simulink model "untitled"  (R2025b)
settings: Solver=VariableStepAuto  StartTime=0.0  StopTime=26  RelTol=1e-3
libraries: neural x35
(part 1 of 2)
settings Model: Creator=Jimmy  LastModifiedBy=Pushkaraj
settings DebuggingCC: UnconnectedInputMsg=warning  UnconnectedOutputMsg=warning  UnconnectedLineMsg=warning
settings ModelReferenceCC: EnableRefExpFcnMdlSchedulingChecks=on
settings RTWCC: GPUComputeCapability=3.5  DLArmComputeVersion=19.05

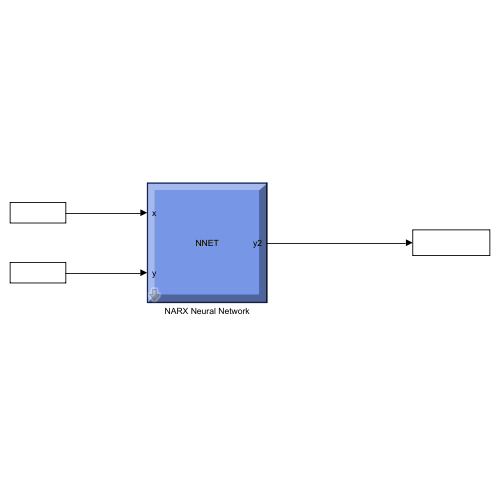
[thumbnail: Simulink's stored preview of the top-level diagram]
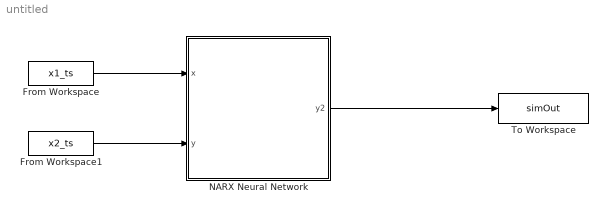
== system untitled ==
  From Workspace : FromWorkspace  VariableName=x1_ts  SampleTime=1  OutputAfterFinalValue=Setting to zero
  From Workspace1 : FromWorkspace  VariableName=x2_ts  SampleTime=1  OutputAfterFinalValue=Setting to zero
  NARX Neural Network : Subsystem  mask{pi_input_1_delayed_1=[0;0;0;0], pi_input_1_delayed_2=[0;0;0;0], pi_input_2_delayed_1=[0;0;0;0;0;0;0;0;0;0], pi_input_2_delayed_2=[0;0;0;0;0;0;0;0;0;0]}
      mask prompts: pi_input_1_delayed_1 "Preprocessed initial input 1 state at timestep 0."; pi_input_1_delayed_2 "Preprocessed initial input 1 state at timestep -1."; pi_input_2_delayed_1 "Preprocessed initial input 2 state at timestep 0."; pi_input_2_delayed_2 "Preprocessed initial input 2 state at timestep -1."
      mask help: NARX Neural Network
      mask Display: e = 0.06;c1 = [120 150 230]/255;c2 = ([120 150 230]+0)/383;c3 = ([120 150 230]+128)/383;patch([0 1 1 0],[0 0 1 1],c1);patch([0 1 1 1-e 1-e 0+e],[0 0 1 1-e 0+e 0+e],c2);patch([0 0 1 1-e 0+e 0+e],[0 1 1 1-e 1-e 0+e],c3);plot([0 1 1 0 0],[0 0 1 1 0]);fprintf('NNET');port_label('input',1,' x');port_label('input',2,' y');port_label('output',1,'y2 ');
  To Workspace : ToWorkspace  VariableName=simOut  SampleTime=-1
  wires:
  From Workspace/1 -> NARX Neural Network/1(x)
  From Workspace1/1 -> NARX Neural Network/2(y)
  NARX Neural Network/1(y2) -> To Workspace/1

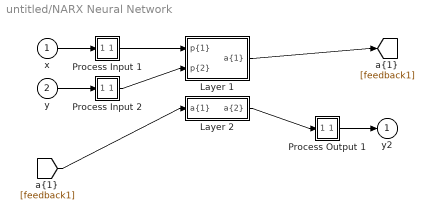
== system untitled/NARX Neural Network ==
  x : Inport  PortDimensions=4  SampleTime=1
      mask Display: e = 0.06;c1 = [120 230 180]/255;c2 = ([120 230 180]+0)/(256+128);c3 = ([120 230 180]+128)/(256+128);patch([0 1 1 0],[0 0 1 1],c1);patch([0 1 1 1-e 1-e 0+e],[0 0 1 1-e 0+e 0+e],c2);patch([0 0 1 1-e 0+e 0+e],[0 1 1 1-e 1-e 0+e],c3);plot([0 1 1 0 0],[0 0 1 1 0]);
  y : Inport  Port=2  PortDimensions=10  SampleTime=1
      mask Display: e = 0.06;c1 = [120 230 180]/255;c2 = ([120 230 180]+0)/(256+128);c3 = ([120 230 180]+128)/(256+128);patch([0 1 1 0],[0 0 1 1],c1);patch([0 1 1 1-e 1-e 0+e],[0 0 1 1-e 0+e 0+e],c2);patch([0 0 1 1-e 0+e 0+e],[0 1 1 1-e 1-e 0+e],c3);plot([0 1 1 0 0],[0 0 1 1 0]);
  Layer 1 : Subsystem
      mask Display: e = 0.06;c1 = [120 150 230]/255;c2 = ([120 150 230]+0)/383;c3 = ([120 150 230]+128)/383;patch([0 1 1 0],[0 0 1 1],c1);patch([0 1 1 1-e 1-e 0+e],[0 0 1 1-e 0+e 0+e],c2);patch([0 0 1 1-e 0+e 0+e],[0 1 1 1-e 1-e 0+e],c3);plot([0 1 1 0 0],[0 0 1 1 0]);
  Layer 2 : Subsystem
      mask Display: e = 0.06;c1 = [120 150 230]/255;c2 = ([120 150 230]+0)/383;c3 = ([120 150 230]+128)/383;patch([0 1 1 0],[0 0 1 1],c1);patch([0 1 1 1-e 1-e 0+e],[0 0 1 1-e 0+e 0+e],c2);patch([0 0 1 1-e 0+e 0+e],[0 1 1 1-e 1-e 0+e],c3);plot([0 1 1 0 0],[0 0 1 1 0]);
  Process Input 1 : Subsystem
      mask Display: e = 0.06;c1 = [120 150 230]/255;c2 = ([120 150 230]+0)/383;c3 = ([120 150 230]+128)/383;patch([0 1 1 0],[0 0 1 1],c1);patch([0 1 1 1-e 1-e 0+e],[0 0 1 1-e 0+e 0+e],c2);patch([0 0 1 1-e 0+e 0+e],[0 1 1 1-e 1-e 0+e],c3);plot([0 1 1 0 0],[0 0 1 1 0]);
  Process Input 2 : Subsystem
      mask Display: e = 0.06;c1 = [120 150 230]/255;c2 = ([120 150 230]+0)/383;c3 = ([120 150 230]+128)/383;patch([0 1 1 0],[0 0 1 1],c1);patch([0 1 1 1-e 1-e 0+e],[0 0 1 1-e 0+e 0+e],c2);patch([0 0 1 1-e 0+e 0+e],[0 1 1 1-e 1-e 0+e],c3);plot([0 1 1 0 0],[0 0 1 1 0]);
  Process Output 1 : Subsystem
      mask Display: e = 0.06;c1 = [120 150 230]/255;c2 = ([120 150 230]+0)/383;c3 = ([120 150 230]+128)/383;patch([0 1 1 0],[0 0 1 1],c1);patch([0 1 1 1-e 1-e 0+e],[0 0 1 1-e 0+e 0+e],c2);patch([0 0 1 1-e 0+e 0+e],[0 1 1 1-e 1-e 0+e],c3);plot([0 1 1 0 0],[0 0 1 1 0]);
  y2 : Outport  InitialOutput=[0;0;0;0;0;0;0;0;0;0]
      mask Display: e = 0.06;c1 = [120 230 180]/255;c2 = ([120 230 180]+0)/(256+128);c3 = ([120 230 180]+128)/(256+128);patch([0 1 1 0],[0 0 1 1],c1);patch([0 1 1 1-e 1-e 0+e],[0 0 1 1-e 0+e 0+e],c2);patch([0 0 1 1-e 0+e 0+e],[0 1 1 1-e 1-e 0+e],c3);plot([0 1 1 0 0],[0 0 1 1 0]);
  wires:
  x/1 -> Process Input 1/1(x)
  y/1 -> Process Input 2/1(x)
  Process Output 1/1(y) -> y2/1
  Process Input 1/1(p) -> Layer 1/1("p{1}")
  Process Input 2/1(p) -> Layer 1/2("p{2}")
  Layer 1/1("a{1}") -> [feedback1]
  [feedback1] -> Layer 2/1("a{1} ")
  Layer 2/1("a{2}") -> Process Output 1/1(a)

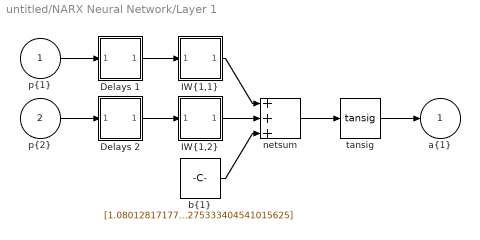
== system untitled/NARX Neural Network/Layer 1 ==
  "p{1}" : Inport  PortDimensions=4  SampleTime=1
      mask Display: e = 0.06;c1 = [120 230 180]/255;c2 = ([120 230 180]+0)/(256+128);c3 = ([120 230 180]+128)/(256+128);patch([0 1 1 0],[0 0 1 1],c1);patch([0 1 1 1-e 1-e 0+e],[0 0 1 1-e 0+e 0+e],c2);patch([0 0 1 1-e 0+e 0+e],[0 1 1 1-e 1-e 0+e],c3);plot([0 1 1 0 0],[0 0 1 1 0]);
  "p{2}" : Inport  Port=2  PortDimensions=10  SampleTime=1
      mask Display: e = 0.06;c1 = [120 230 180]/255;c2 = ([120 230 180]+0)/(256+128);c3 = ([120 230 180]+128)/(256+128);patch([0 1 1 0],[0 0 1 1],c1);patch([0 1 1 1-e 1-e 0+e],[0 0 1 1-e 0+e 0+e],c2);patch([0 0 1 1-e 0+e 0+e],[0 1 1 1-e 1-e 0+e],c3);plot([0 1 1 0 0],[0 0 1 1 0]);
  Delays 1 : Subsystem
      mask Display: e = 0.06;c1 = [120 150 230]/255;c2 = ([120 150 230]+0)/383;c3 = ([120 150 230]+128)/383;patch([0 1 1 0],[0 0 1 1],c1);patch([0 1 1 1-e 1-e 0+e],[0 0 1 1-e 0+e 0+e],c2);patch([0 0 1 1-e 0+e 0+e],[0 1 1 1-e 1-e 0+e],c3);plot([0 1 1 0 0],[0 0 1 1 0]);disp('1-2');
  Delays 2 : Subsystem
      mask Display: e = 0.06;c1 = [120 150 230]/255;c2 = ([120 150 230]+0)/383;c3 = ([120 150 230]+128)/383;patch([0 1 1 0],[0 0 1 1],c1);patch([0 1 1 1-e 1-e 0+e],[0 0 1 1-e 0+e 0+e],c2);patch([0 0 1 1-e 0+e 0+e],[0 1 1 1-e 1-e 0+e],c3);plot([0 1 1 0 0],[0 0 1 1 0]);disp('1-2');
  "IW{1,1}" : Subsystem
      mask Display: e = 0.06;c1 = [120 150 230]/255;c2 = ([120 150 230]+0)/383;c3 = ([120 150 230]+128)/383;patch([0 1 1 0],[0 0 1 1],c1);patch([0 1 1 1-e 1-e 0+e],[0 0 1 1-e 0+e 0+e],c2);patch([0 0 1 1-e 0+e 0+e],[0 1 1 1-e 1-e 0+e],c3);plot([0 1 1 0 0],[0 0 1 1 0]);disp('W');
  "IW{1,2}" : Subsystem
      mask Display: e = 0.06;c1 = [120 150 230]/255;c2 = ([120 150 230]+0)/383;c3 = ([120 150 230]+128)/383;patch([0 1 1 0],[0 0 1 1],c1);patch([0 1 1 1-e 1-e 0+e],[0 0 1 1-e 0+e 0+e],c2);patch([0 0 1 1-e 0+e 0+e],[0 1 1 1-e 1-e 0+e],c3);plot([0 1 1 0 0],[0 0 1 1 0]);disp('W');
  "b{1}" : Constant  Value=[1.0801281717727395648154242735472507774829864501953125;-1.310912600446497489059538565925322473049163818359375;0.9404335907148200224270340186194516718387603759765625;-0.81368279707896140617862101862556301057338714599609375;0.432949116587421134472180028751608915627002716064453125;0.068784327532554534467834628230775706470012664794921875;-0.29264096087120716749296889247489161789417266845703125;0.7805557229172677136119773422251455485820770263671875;-1.12796688888643092951724611339159309864044189453125;1.7338922757099712868011920363642275333404541015625]
      mask Display: e = 0.06;c1 = [120 150 230]/255;c2 = ([120 150 230]+0)/383;c3 = ([120 150 230]+128)/383;patch([0 1 1 0],[0 0 1 1],c1);patch([0 1 1 1-e 1-e 0+e],[0 0 1 1-e 0+e 0+e],c2);patch([0 0 1 1-e 0+e 0+e],[0 1 1 1-e 1-e 0+e],c3);plot([0 1 1 0 0],[0 0 1 1 0]);disp('b');
  netsum : Sum  Inputs=3  InputSameDT=on  SaturateOnIntegerOverflow=on  OutDataTypeStr=Inherit: Same as first input
      mask Display: e = 0.06;c1 = [120 150 230]/255;c2 = ([120 150 230]+0)/383;c3 = ([120 150 230]+128)/383;patch([0 1 1 0],[0 0 1 1],c1);patch([0 1 1 1-e 1-e 0+e],[0 0 1 1-e 0+e 0+e],c2);patch([0 0 1 1-e 0+e 0+e],[0 1 1 1-e 1-e 0+e],c3);plot([0 1 1 0 0],[0 0 1 1 0]);disp('+');
  tansig : neural/Transfer Functions/tansig
  "a{1}" : Outport  InitialOutput=[0;0;0;0;0;0;0;0;0;0]
      mask Display: e = 0.06;c1 = [120 230 180]/255;c2 = ([120 230 180]+0)/(256+128);c3 = ([120 230 180]+128)/(256+128);patch([0 1 1 0],[0 0 1 1],c1);patch([0 1 1 1-e 1-e 0+e],[0 0 1 1-e 0+e 0+e],c2);patch([0 0 1 1-e 0+e 0+e],[0 1 1 1-e 1-e 0+e],c3);plot([0 1 1 0 0],[0 0 1 1 0]);
  wires:
  "p{1}"/1 -> Delays 1/1("p{1}")
  Delays 1/1("pd{1,1}") -> "IW{1,1}"/1("pd{1,1}")
  "IW{1,1}"/1("iz{1,1}") -> netsum/1
  "p{2}"/1 -> Delays 2/1("p{1}")
  Delays 2/1("pd{1,2}") -> "IW{1,2}"/1("pd{1,2}")
  "IW{1,2}"/1("iz{1,2}") -> netsum/2
  "b{1}"/1 -> netsum/3
  netsum/1 -> tansig/1
  tansig/1 -> "a{1}"/1

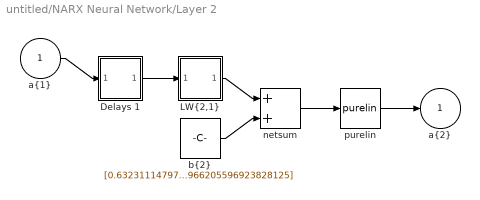
== system untitled/NARX Neural Network/Layer 2 ==
  "a{1} " : Inport  PortDimensions=10  SampleTime=1
      mask Display: e = 0.06;c1 = [120 230 180]/255;c2 = ([120 230 180]+0)/(256+128);c3 = ([120 230 180]+128)/(256+128);patch([0 1 1 0],[0 0 1 1],c1);patch([0 1 1 1-e 1-e 0+e],[0 0 1 1-e 0+e 0+e],c2);patch([0 0 1 1-e 0+e 0+e],[0 1 1 1-e 1-e 0+e],c3);plot([0 1 1 0 0],[0 0 1 1 0]);
  Delays 1 : Subsystem
      mask Display: e = 0.06;c1 = [120 150 230]/255;c2 = ([120 150 230]+0)/383;c3 = ([120 150 230]+128)/383;patch([0 1 1 0],[0 0 1 1],c1);patch([0 1 1 1-e 1-e 0+e],[0 0 1 1-e 0+e 0+e],c2);patch([0 0 1 1-e 0+e 0+e],[0 1 1 1-e 1-e 0+e],c3);plot([0 1 1 0 0],[0 0 1 1 0]);disp('0');
  "LW{2,1}" : Subsystem
      mask Display: e = 0.06;c1 = [120 150 230]/255;c2 = ([120 150 230]+0)/383;c3 = ([120 150 230]+128)/383;patch([0 1 1 0],[0 0 1 1],c1);patch([0 1 1 1-e 1-e 0+e],[0 0 1 1-e 0+e 0+e],c2);patch([0 0 1 1-e 0+e 0+e],[0 1 1 1-e 1-e 0+e],c3);plot([0 1 1 0 0],[0 0 1 1 0]);disp('W');
  "b{2}" : Constant  Value=[0.63231114797012033523770924148266203701496124267578125;0.077425009453641446821592353444430045783519744873046875;0.69336797498678903739488532664836384356021881103515625;0.96191102890088908683452473269426263868808746337890625;-0.01280570802179627383499127546429008361883461475372314453125;0.1820181237505598959014463389394222758710384368896484375;-3.18169363647799041672215025755576789379119873046875;-0.374160373721601657859281431228737346827983856201171875;-0.778234975833982378645714561571367084980010986328125;0.8437778280262862029559300935943610966205596923828125]
      mask Display: e = 0.06;c1 = [120 150 230]/255;c2 = ([120 150 230]+0)/383;c3 = ([120 150 230]+128)/383;patch([0 1 1 0],[0 0 1 1],c1);patch([0 1 1 1-e 1-e 0+e],[0 0 1 1-e 0+e 0+e],c2);patch([0 0 1 1-e 0+e 0+e],[0 1 1 1-e 1-e 0+e],c3);plot([0 1 1 0 0],[0 0 1 1 0]);disp('b');
  netsum : Sum  Inputs=2  InputSameDT=on  SaturateOnIntegerOverflow=on  OutDataTypeStr=Inherit: Same as first input
      mask Display: e = 0.06;c1 = [120 150 230]/255;c2 = ([120 150 230]+0)/383;c3 = ([120 150 230]+128)/383;patch([0 1 1 0],[0 0 1 1],c1);patch([0 1 1 1-e 1-e 0+e],[0 0 1 1-e 0+e 0+e],c2);patch([0 0 1 1-e 0+e 0+e],[0 1 1 1-e 1-e 0+e],c3);plot([0 1 1 0 0],[0 0 1 1 0]);disp('+');
  purelin : neural/Transfer Functions/purelin
  "a{2}" : Outport  InitialOutput=[0;0;0;0;0;0;0;0;0;0]
      mask Display: e = 0.06;c1 = [120 230 180]/255;c2 = ([120 230 180]+0)/(256+128);c3 = ([120 230 180]+128)/(256+128);patch([0 1 1 0],[0 0 1 1],c1);patch([0 1 1 1-e 1-e 0+e],[0 0 1 1-e 0+e 0+e],c2);patch([0 0 1 1-e 0+e 0+e],[0 1 1 1-e 1-e 0+e],c3);plot([0 1 1 0 0],[0 0 1 1 0]);
  wires:
  "a{1} "/1 -> Delays 1/1("p{2}")
  Delays 1/1("pd{2,1}") -> "LW{2,1}"/1("ad{2,1}")
  "LW{2,1}"/1("lz{2,1}") -> netsum/1
  "b{2}"/1 -> netsum/2
  netsum/1 -> purelin/1
  purelin/1 -> "a{2}"/1

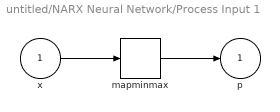
== system untitled/NARX Neural Network/Process Input 1 ==
  x : Inport  PortDimensions=4  SampleTime=1
      mask Display: e = 0.06;c1 = [120 230 180]/255;c2 = ([120 230 180]+0)/(256+128);c3 = ([120 230 180]+128)/(256+128);patch([0 1 1 0],[0 0 1 1],c1);patch([0 1 1 1-e 1-e 0+e],[0 0 1 1-e 0+e 0+e],c2);patch([0 0 1 1-e 0+e 0+e],[0 1 1 1-e 1-e 0+e],c3);plot([0 1 1 0 0],[0 0 1 1 0]);
  mapminmax : neural/Processing Functions/mapminmax  xmin=[0;-4.44000000000000039079850466806;0;0]  xmax=[81;3.33000000000000007105427357601;354;168]  ymin=-1  ymax=1
  p : Outport  PortDimensions=4  SampleTime=1
      mask Display: e = 0.06;c1 = [120 230 180]/255;c2 = ([120 230 180]+0)/(256+128);c3 = ([120 230 180]+128)/(256+128);patch([0 1 1 0],[0 0 1 1],c1);patch([0 1 1 1-e 1-e 0+e],[0 0 1 1-e 0+e 0+e],c2);patch([0 0 1 1-e 0+e 0+e],[0 1 1 1-e 1-e 0+e],c3);plot([0 1 1 0 0],[0 0 1 1 0]);
  wires:
  x/1 -> mapminmax/1
  mapminmax/1 -> p/1

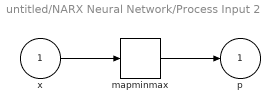
== system untitled/NARX Neural Network/Process Input 2 ==
  x : Inport  PortDimensions=10  SampleTime=1
      mask Display: e = 0.06;c1 = [120 230 180]/255;c2 = ([120 230 180]+0)/(256+128);c3 = ([120 230 180]+128)/(256+128);patch([0 1 1 0],[0 0 1 1],c1);patch([0 1 1 1-e 1-e 0+e],[0 0 1 1-e 0+e 0+e],c2);patch([0 0 1 1-e 0+e 0+e],[0 1 1 1-e 1-e 0+e],c3);plot([0 1 1 0 0],[0 0 1 1 0]);
  mapminmax : neural/Processing Functions/mapminmax  xmin=[0;0;0;0;0;0;0;0;0;0]  xmax=[1;1;1;1;1;1;1;1;1;1]  ymin=-1  ymax=1
  p : Outport  PortDimensions=10  SampleTime=1
      mask Display: e = 0.06;c1 = [120 230 180]/255;c2 = ([120 230 180]+0)/(256+128);c3 = ([120 230 180]+128)/(256+128);patch([0 1 1 0],[0 0 1 1],c1);patch([0 1 1 1-e 1-e 0+e],[0 0 1 1-e 0+e 0+e],c2);patch([0 0 1 1-e 0+e 0+e],[0 1 1 1-e 1-e 0+e],c3);plot([0 1 1 0 0],[0 0 1 1 0]);
  wires:
  x/1 -> mapminmax/1
  mapminmax/1 -> p/1

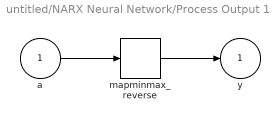
== system untitled/NARX Neural Network/Process Output 1 ==
  a : Inport  PortDimensions=10  SampleTime=1
      mask Display: e = 0.06;c1 = [120 230 180]/255;c2 = ([120 230 180]+0)/(256+128);c3 = ([120 230 180]+128)/(256+128);patch([0 1 1 0],[0 0 1 1],c1);patch([0 1 1 1-e 1-e 0+e],[0 0 1 1-e 0+e 0+e],c2);patch([0 0 1 1-e 0+e 0+e],[0 1 1 1-e 1-e 0+e],c3);plot([0 1 1 0 0],[0 0 1 1 0]);
  mapminmax_reverse : neural/Processing Functions/mapminmax_reverse  xmin=[0;0;0;0;0;0;0;0;0;0]  xmax=[1;1;1;1;1;1;1;1;1;1]  ymin=-1  ymax=1
  y : Outport  PortDimensions=10  SampleTime=1
      mask Display: e = 0.06;c1 = [120 230 180]/255;c2 = ([120 230 180]+0)/(256+128);c3 = ([120 230 180]+128)/(256+128);patch([0 1 1 0],[0 0 1 1],c1);patch([0 1 1 1-e 1-e 0+e],[0 0 1 1-e 0+e 0+e],c2);patch([0 0 1 1-e 0+e 0+e],[0 1 1 1-e 1-e 0+e],c3);plot([0 1 1 0 0],[0 0 1 1 0]);
  wires:
  a/1 -> mapminmax_reverse/1
  mapminmax_reverse/1 -> y/1

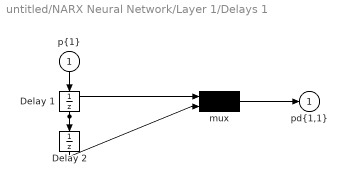
== system untitled/NARX Neural Network/Layer 1/Delays 1 ==
  "p{1}" : Inport  PortDimensions=4  SampleTime=1
      mask Display: e = 0.06;c1 = [120 230 180]/255;c2 = ([120 230 180]+0)/(256+128);c3 = ([120 230 180]+128)/(256+128);patch([0 1 1 0],[0 0 1 1],c1);patch([0 1 1 1-e 1-e 0+e],[0 0 1 1-e 0+e 0+e],c2);patch([0 0 1 1-e 0+e 0+e],[0 1 1 1-e 1-e 0+e],c3);plot([0 1 1 0 0],[0 0 1 1 0]);
  Delay 1 : UnitDelay  InitialCondition=pi_input_1_delayed_1
      mask Display: e = 0.06;c1 = [120 150 230]/255;c2 = ([120 150 230]+0)/383;c3 = ([120 150 230]+128)/383;patch([0 1 1 0],[0 0 1 1],c1);patch([0 1 1 1-e 1-e 0+e],[0 0 1 1-e 0+e 0+e],c2);patch([0 0 1 1-e 0+e 0+e],[0 1 1 1-e 1-e 0+e],c3);plot([0 1 1 0 0],[0 0 1 1 0]);disp('D')
  Delay 2 : UnitDelay  InitialCondition=pi_input_1_delayed_2
      mask Display: e = 0.06;c1 = [120 150 230]/255;c2 = ([120 150 230]+0)/383;c3 = ([120 150 230]+128)/383;patch([0 1 1 0],[0 0 1 1],c1);patch([0 1 1 1-e 1-e 0+e],[0 0 1 1-e 0+e 0+e],c2);patch([0 0 1 1-e 0+e 0+e],[0 1 1 1-e 1-e 0+e],c3);plot([0 1 1 0 0],[0 0 1 1 0]);disp('D')
  mux : Mux  Inputs=2
      mask Display: e = 0.06;c1 = [120 150 230]/255;c2 = ([120 150 230]+0)/383;c3 = ([120 150 230]+128)/383;patch([0 1 1 0],[0 0 1 1],c1);patch([0 1 1 1-e 1-e 0+e],[0 0 1 1-e 0+e 0+e],c2);patch([0 0 1 1-e 0+e 0+e],[0 1 1 1-e 1-e 0+e],c3);plot([0 1 1 0 0],[0 0 1 1 0]);disp('Mux')
  "pd{1,1}" : Outport
      mask Display: e = 0.06;c1 = [120 230 180]/255;c2 = ([120 230 180]+0)/(256+128);c3 = ([120 230 180]+128)/(256+128);patch([0 1 1 0],[0 0 1 1],c1);patch([0 1 1 1-e 1-e 0+e],[0 0 1 1-e 0+e 0+e],c2);patch([0 0 1 1-e 0+e 0+e],[0 1 1 1-e 1-e 0+e],c3);plot([0 1 1 0 0],[0 0 1 1 0]);
  wires:
  "p{1}"/1 -> Delay 1/1
  Delay 1/1 -> Delay 2/1, mux/1
  Delay 2/1 -> mux/2
  mux/1 -> "pd{1,1}"/1

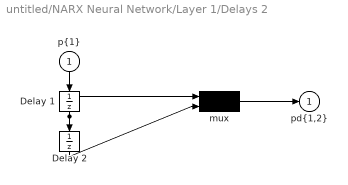
== system untitled/NARX Neural Network/Layer 1/Delays 2 ==
  "p{1}" : Inport  PortDimensions=10  SampleTime=1
      mask Display: e = 0.06;c1 = [120 230 180]/255;c2 = ([120 230 180]+0)/(256+128);c3 = ([120 230 180]+128)/(256+128);patch([0 1 1 0],[0 0 1 1],c1);patch([0 1 1 1-e 1-e 0+e],[0 0 1 1-e 0+e 0+e],c2);patch([0 0 1 1-e 0+e 0+e],[0 1 1 1-e 1-e 0+e],c3);plot([0 1 1 0 0],[0 0 1 1 0]);
  Delay 1 : UnitDelay  InitialCondition=pi_input_2_delayed_1
      mask Display: e = 0.06;c1 = [120 150 230]/255;c2 = ([120 150 230]+0)/383;c3 = ([120 150 230]+128)/383;patch([0 1 1 0],[0 0 1 1],c1);patch([0 1 1 1-e 1-e 0+e],[0 0 1 1-e 0+e 0+e],c2);patch([0 0 1 1-e 0+e 0+e],[0 1 1 1-e 1-e 0+e],c3);plot([0 1 1 0 0],[0 0 1 1 0]);disp('D')
  Delay 2 : UnitDelay  InitialCondition=pi_input_2_delayed_2
      mask Display: e = 0.06;c1 = [120 150 230]/255;c2 = ([120 150 230]+0)/383;c3 = ([120 150 230]+128)/383;patch([0 1 1 0],[0 0 1 1],c1);patch([0 1 1 1-e 1-e 0+e],[0 0 1 1-e 0+e 0+e],c2);patch([0 0 1 1-e 0+e 0+e],[0 1 1 1-e 1-e 0+e],c3);plot([0 1 1 0 0],[0 0 1 1 0]);disp('D')
  mux : Mux  Inputs=2
      mask Display: e = 0.06;c1 = [120 150 230]/255;c2 = ([120 150 230]+0)/383;c3 = ([120 150 230]+128)/383;patch([0 1 1 0],[0 0 1 1],c1);patch([0 1 1 1-e 1-e 0+e],[0 0 1 1-e 0+e 0+e],c2);patch([0 0 1 1-e 0+e 0+e],[0 1 1 1-e 1-e 0+e],c3);plot([0 1 1 0 0],[0 0 1 1 0]);disp('Mux')
  "pd{1,2}" : Outport
      mask Display: e = 0.06;c1 = [120 230 180]/255;c2 = ([120 230 180]+0)/(256+128);c3 = ([120 230 180]+128)/(256+128);patch([0 1 1 0],[0 0 1 1],c1);patch([0 1 1 1-e 1-e 0+e],[0 0 1 1-e 0+e 0+e],c2);patch([0 0 1 1-e 0+e 0+e],[0 1 1 1-e 1-e 0+e],c3);plot([0 1 1 0 0],[0 0 1 1 0]);
  wires:
  "p{1}"/1 -> Delay 1/1
  Delay 1/1 -> Delay 2/1, mux/1
  Delay 2/1 -> mux/2
  mux/1 -> "pd{1,2}"/1

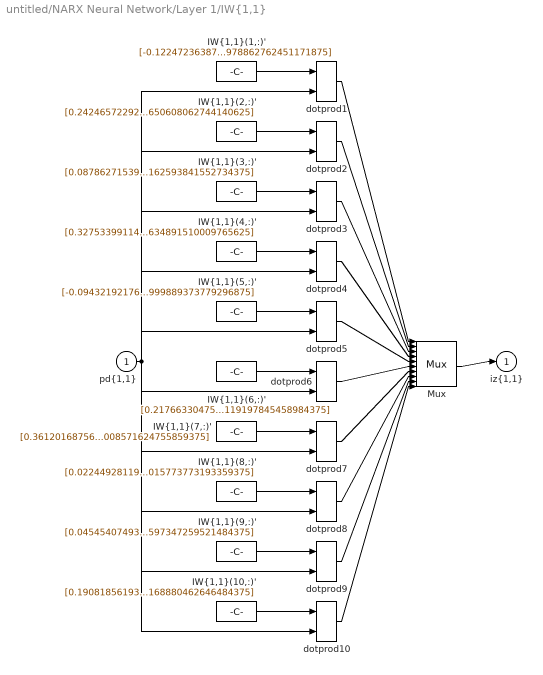
== system untitled/NARX Neural Network/Layer 1/IW{1,1} ==
  "pd{1,1}" : Inport  PortDimensions=8  SampleTime=1
      mask Display: e = 0.06;c1 = [120 230 180]/255;c2 = ([120 230 180]+0)/(256+128);c3 = ([120 230 180]+128)/(256+128);patch([0 1 1 0],[0 0 1 1],c1);patch([0 1 1 1-e 1-e 0+e],[0 0 1 1-e 0+e 0+e],c2);patch([0 0 1 1-e 0+e 0+e],[0 1 1 1-e 1-e 0+e],c3);plot([0 1 1 0 0],[0 0 1 1 0]);
  "IW{1,1}(1,:)'" : Constant  Value=[-0.1224723638716402052128984223600127734243869781494140625;-0.3272459825504128172468654156546108424663543701171875;-0.1644271449580847199722910545460763387382030487060546875;0.57264450002805056261223626279388554394245147705078125;-0.06048568878075073762534685783975874073803424835205078125;0.223227164473066286287661341702914796769618988037109375;-0.019058424240247777425860675748481298796832561492919921875;0.546018070579335823566680119256488978862762451171875]
      mask Display: e = 0.06;c1 = [120 150 230]/255;c2 = ([120 150 230]+0)/383;c3 = ([120 150 230]+128)/383;patch([0 1 1 0],[0 0 1 1],c1);patch([0 1 1 1-e 1-e 0+e],[0 0 1 1-e 0+e 0+e],c2);patch([0 0 1 1-e 0+e 0+e],[0 1 1 1-e 1-e 0+e],c3);plot([0 1 1 0 0],[0 0 1 1 0]);disp('Weights');
  "IW{1,1}(10,:)'" : Constant  Value=[0.1908185619389482223784426651036483235657215118408203125;-0.364308552820070408184705001986003480851650238037109375;0.042247088415687049367530647714374936185777187347412109375;-0.4511925818793398601513899848214350640773773193359375;0.2259289495251827484256779143834137357771396636962890625;-0.3262510626149310866139785503037273883819580078125;-0.0550061423234808055671152260401868261396884918212890625;-0.2441178010327449410254985195933841168880462646484375]
      mask Display: e = 0.06;c1 = [120 150 230]/255;c2 = ([120 150 230]+0)/383;c3 = ([120 150 230]+128)/383;patch([0 1 1 0],[0 0 1 1],c1);patch([0 1 1 1-e 1-e 0+e],[0 0 1 1-e 0+e 0+e],c2);patch([0 0 1 1-e 0+e 0+e],[0 1 1 1-e 1-e 0+e],c3);plot([0 1 1 0 0],[0 0 1 1 0]);disp('Weights');
  "IW{1,1}(2,:)'" : Constant  Value=[0.2424657229293740723363725919625721871852874755859375;0.61044817882070490089319036997039802372455596923828125;0.029426927959954295166422610918743885122239589691162109375;-0.389312569909250838495751168011338450014591217041015625;-0.362729002225335772635617104242555797100067138671875;-0.2394230697254556561315297358305542729794979095458984375;-0.068311785910934952337214554063393734395503997802734375;-0.0726366665121031263030459967922070063650608062744140625]
      mask Display: e = 0.06;c1 = [120 150 230]/255;c2 = ([120 150 230]+0)/383;c3 = ([120 150 230]+128)/383;patch([0 1 1 0],[0 0 1 1],c1);patch([0 1 1 1-e 1-e 0+e],[0 0 1 1-e 0+e 0+e],c2);patch([0 0 1 1-e 0+e 0+e],[0 1 1 1-e 1-e 0+e],c3);plot([0 1 1 0 0],[0 0 1 1 0]);disp('Weights');
  "IW{1,1}(3,:)'" : Constant  Value=[0.0878627153945485683816940536416950635612010955810546875;-0.10868956786818624593582427451110561378300189971923828125;0.003320688322202099661273333452982114977203309535980224609375;-0.028863266432759278334874153415512409992516040802001953125;-0.004309564181281520280075714168788181268610060214996337890625;0.093685284602520735308672783503425307571887969970703125;-0.0385581469925005693166752962497412227094173431396484375;0.08545928123295985778806738153434707783162593841552734375]
      mask Display: e = 0.06;c1 = [120 150 230]/255;c2 = ([120 150 230]+0)/383;c3 = ([120 150 230]+128)/383;patch([0 1 1 0],[0 0 1 1],c1);patch([0 1 1 1-e 1-e 0+e],[0 0 1 1-e 0+e 0+e],c2);patch([0 0 1 1-e 0+e 0+e],[0 1 1 1-e 1-e 0+e],c3);plot([0 1 1 0 0],[0 0 1 1 0]);disp('Weights');
  "IW{1,1}(4,:)'" : Constant  Value=[0.32753399114338510589305997200426645576953887939453125;-0.06516688941377120347642204478688654489815235137939453125;0.2778103137181517912068784426082856953144073486328125;0.538106050871987928729822669993154704570770263671875;0.269643477419196420097335931131965480744838714599609375;0.1808721157042202654086082702633575536310672760009765625;-0.20367457353888440696465522705693729221820831298828125;0.1079168278560746208061260631438926793634891510009765625]
      mask Display: e = 0.06;c1 = [120 150 230]/255;c2 = ([120 150 230]+0)/383;c3 = ([120 150 230]+128)/383;patch([0 1 1 0],[0 0 1 1],c1);patch([0 1 1 1-e 1-e 0+e],[0 0 1 1-e 0+e 0+e],c2);patch([0 0 1 1-e 0+e 0+e],[0 1 1 1-e 1-e 0+e],c3);plot([0 1 1 0 0],[0 0 1 1 0]);disp('Weights');
  "IW{1,1}(5,:)'" : Constant  Value=[-0.09432192176716279463644099223529337905347347259521484375;0.384912230366909413614706636508344672620296478271484375;-0.013107624645180011857537039077215013094246387481689453125;0.432402225644634763401796817561262287199497222900390625;0.01467470846526797330355851300964786787517368793487548828125;-0.311855250125882499379059709099237807095050811767578125;0.007566019275313939397575868639478358090855181217193603515625;0.35924302483212766645692681777290999889373779296875]
      mask Display: e = 0.06;c1 = [120 150 230]/255;c2 = ([120 150 230]+0)/383;c3 = ([120 150 230]+128)/383;patch([0 1 1 0],[0 0 1 1],c1);patch([0 1 1 1-e 1-e 0+e],[0 0 1 1-e 0+e 0+e],c2);patch([0 0 1 1-e 0+e 0+e],[0 1 1 1-e 1-e 0+e],c3);plot([0 1 1 0 0],[0 0 1 1 0]);disp('Weights');
  "IW{1,1}(6,:)'" : Constant  Value=[0.217663304750638719742283910818514414131641387939453125;0.0160955223635426032668949147819148492999374866485595703125;0.03373270263645840316701907113383640535175800323486328125;0.461161766861531818850750141791650094091892242431640625;-0.1841467185569863052041483797438559122383594512939453125;-0.06357475733769908654569036343673360534012317657470703125;-0.041177180544662406180833613689173944294452667236328125;0.0034308485870010846895128420186438233940862119197845458984375]
      mask Display: e = 0.06;c1 = [120 150 230]/255;c2 = ([120 150 230]+0)/383;c3 = ([120 150 230]+128)/383;patch([0 1 1 0],[0 0 1 1],c1);patch([0 1 1 1-e 1-e 0+e],[0 0 1 1-e 0+e 0+e],c2);patch([0 0 1 1-e 0+e 0+e],[0 1 1 1-e 1-e 0+e],c3);plot([0 1 1 0 0],[0 0 1 1 0]);disp('Weights');
  "IW{1,1}(7,:)'" : Constant  Value=[0.36120168756955084443660553006338886916637420654296875;-0.1693601286070866851485305915048229508101940155029296875;-0.037610779283216357049557387881577596999704837799072265625;-0.2152776354201784148045817346428520977497100830078125;0.06378422228839415730750062039078329689800739288330078125;0.07441943145178138430129166636106674559414386749267578125;-0.0062424893192859591539711772156806546263396739959716796875;-0.129242141700021517802809967179200612008571624755859375]
      mask Display: e = 0.06;c1 = [120 150 230]/255;c2 = ([120 150 230]+0)/383;c3 = ([120 150 230]+128)/383;patch([0 1 1 0],[0 0 1 1],c1);patch([0 1 1 1-e 1-e 0+e],[0 0 1 1-e 0+e 0+e],c2);patch([0 0 1 1-e 0+e 0+e],[0 1 1 1-e 1-e 0+e],c3);plot([0 1 1 0 0],[0 0 1 1 0]);disp('Weights');
  "IW{1,1}(8,:)'" : Constant  Value=[0.0224492811909891530619542976410230039618909358978271484375;0.004359173224923172142164506936978796147741377353668212890625;-0.0123879902387121453022356121209668344818055629730224609375;0.261814032696891130225225197136751376092433929443359375;-0.00952574033227335074947017545810012961737811565399169921875;0.1042534958370524289517078386779758147895336151123046875;0.009669143693752720036815873072555405087769031524658203125;0.00382504692234129917149942912146798335015773773193359375]
      mask Display: e = 0.06;c1 = [120 150 230]/255;c2 = ([120 150 230]+0)/383;c3 = ([120 150 230]+128)/383;patch([0 1 1 0],[0 0 1 1],c1);patch([0 1 1 1-e 1-e 0+e],[0 0 1 1-e 0+e 0+e],c2);patch([0 0 1 1-e 0+e 0+e],[0 1 1 1-e 1-e 0+e],c3);plot([0 1 1 0 0],[0 0 1 1 0]);disp('Weights');
  "IW{1,1}(9,:)'" : Constant  Value=[0.045454074938318156373640022138715721666812896728515625;0.43299066027697208358659963778336532413959503173828125;-0.07572779606926942352895792964773136191070079803466796875;0.297556185334404366127358798621571622788906097412109375;-0.0690048253928155219671936038139392621815204620361328125;-0.345115340545246784831334707632777281105518341064453125;0.1791996384983501056087362712787580676376819610595703125;0.26485060102794777403545367633341811597347259521484375]
      mask Display: e = 0.06;c1 = [120 150 230]/255;c2 = ([120 150 230]+0)/383;c3 = ([120 150 230]+128)/383;patch([0 1 1 0],[0 0 1 1],c1);patch([0 1 1 1-e 1-e 0+e],[0 0 1 1-e 0+e 0+e],c2);patch([0 0 1 1-e 0+e 0+e],[0 1 1 1-e 1-e 0+e],c3);plot([0 1 1 0 0],[0 0 1 1 0]);disp('Weights');
  Mux : Mux  Inputs=10
      mask Display: e = 0.06;c1 = [120 150 230]/255;c2 = ([120 150 230]+0)/383;c3 = ([120 150 230]+128)/383;patch([0 1 1 0],[0 0 1 1],c1);patch([0 1 1 1-e 1-e 0+e],[0 0 1 1-e 0+e 0+e],c2);patch([0 0 1 1-e 0+e 0+e],[0 1 1 1-e 1-e 0+e],c3);plot([0 1 1 0 0],[0 0 1 1 0]);disp('Mux');
  dotprod{1..10} (10 alike) : neural/Weight Functions/dotprod
  "iz{1,1}" : Outport
      mask Display: e = 0.06;c1 = [120 230 180]/255;c2 = ([120 230 180]+0)/(256+128);c3 = ([120 230 180]+128)/(256+128);patch([0 1 1 0],[0 0 1 1],c1);patch([0 1 1 1-e 1-e 0+e],[0 0 1 1-e 0+e 0+e],c2);patch([0 0 1 1-e 0+e 0+e],[0 1 1 1-e 1-e 0+e],c3);plot([0 1 1 0 0],[0 0 1 1 0]);
  wires:
  "IW{1,1}(1,:)'"/1 -> dotprod1/1
  "pd{1,1}"/1 -> dotprod1/2, dotprod2/2, dotprod3/2, dotprod4/2, dotprod5/2, dotprod6/2, dotprod7/2, dotprod8/2, dotprod9/2, dotprod10/2
  dotprod1/1 -> Mux/1
  "IW{1,1}(2,:)'"/1 -> dotprod2/1
  dotprod2/1 -> Mux/2
  "IW{1,1}(3,:)'"/1 -> dotprod3/1
  dotprod3/1 -> Mux/3
  "IW{1,1}(4,:)'"/1 -> dotprod4/1
  dotprod4/1 -> Mux/4
  "IW{1,1}(5,:)'"/1 -> dotprod5/1
  dotprod5/1 -> Mux/5
  "IW{1,1}(6,:)'"/1 -> dotprod6/1
  dotprod6/1 -> Mux/6
  "IW{1,1}(7,:)'"/1 -> dotprod7/1
  dotprod7/1 -> Mux/7
  "IW{1,1}(8,:)'"/1 -> dotprod8/1
  dotprod8/1 -> Mux/8
  "IW{1,1}(9,:)'"/1 -> dotprod9/1
  dotprod9/1 -> Mux/9
  "IW{1,1}(10,:)'"/1 -> dotprod10/1
  dotprod10/1 -> Mux/10
  Mux/1 -> "iz{1,1}"/1

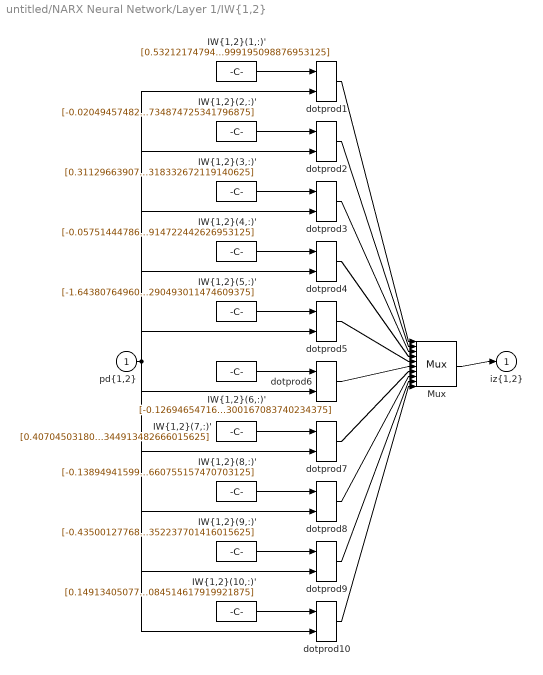
== system untitled/NARX Neural Network/Layer 1/IW{1,2} ==
  "pd{1,2}" : Inport  PortDimensions=20  SampleTime=1
      mask Display: e = 0.06;c1 = [120 230 180]/255;c2 = ([120 230 180]+0)/(256+128);c3 = ([120 230 180]+128)/(256+128);patch([0 1 1 0],[0 0 1 1],c1);patch([0 1 1 1-e 1-e 0+e],[0 0 1 1-e 0+e 0+e],c2);patch([0 0 1 1-e 0+e 0+e],[0 1 1 1-e 1-e 0+e],c3);plot([0 1 1 0 0],[0 0 1 1 0]);
  "IW{1,2}(1,:)'" : Constant  Value=[0.53212174794800748411915947144734673202037811279296875;0.817018572346948968032620541634969413280487060546875;-0.07493102459351637378848209891657461412250995635986328125;0.53944162567220654835864479537121951580047607421875;0.10845896887198758218318062063190154731273651123046875;1.132252522673124150998091863584704697132110595703125;0.327636360657517611283395808641216717660427093505859375;0.70994173397534010572229590252391062676906585693359375;0.5847090073265535092872369204997085034847259521484375;0.522602500198308117518308790749870240688323974609375;0.72376531811480038225425914788502268493175506591796875;0.1984043917971633208541248905021348036825656890869140625;0.59422533919091902188114318050793372094631195068359375;0.478785746744103957173166463689994998276233673095703125;0.57315091609280255369185397285036742687225341796875;0.99686198383266788614065490037319250404834747314453125;0.043988644397989336287668749037038651295006275177001953125;-0.0758886279541541586279862485753255896270275115966796875;0.317474607493858640427930595251382328569889068603515625;0.2195904562016906258481441227559116668999195098876953125]
      mask Display: e = 0.06;c1 = [120 150 230]/255;c2 = ([120 150 230]+0)/383;c3 = ([120 150 230]+128)/383;patch([0 1 1 0],[0 0 1 1],c1);patch([0 1 1 1-e 1-e 0+e],[0 0 1 1-e 0+e 0+e],c2);patch([0 0 1 1-e 0+e 0+e],[0 1 1 1-e 1-e 0+e],c3);plot([0 1 1 0 0],[0 0 1 1 0]);disp('Weights');
  "IW{1,2}(10,:)'" : Constant  Value=[0.149134050770307780009460429937462322413921356201171875;0.016092934597212338321270408414420671761035919189453125;-0.497056507890472010213755993390805087983608245849609375;-0.47348819318803136990680968665401451289653778076171875;0.01510195472959737460205698056370238191448152065277099609375;-0.182922680974307194645689378376118838787078857421875;-0.341974178913040827154645739938132464885711669921875;0.1378741509415832011686831037877709604799747467041015625;-0.38400401242187853778631279055844061076641082763671875;-0.256289846136677823551508481614291667938232421875;-0.462174969453290340748452535990509204566478729248046875;-0.40550556407280946569215984709444455802440643310546875;-0.455556541505276080261666038495604880154132843017578125;-0.60706695608606775493854001979343593120574951171875;0.161792458499850966280320108126034028828144073486328125;0.171043172930342546322890484589152038097381591796875;-0.2160438333158184176507887741536251269280910491943359375;-0.2246726112300536370991466128543834201991558074951171875;-0.1709689141764914876997494275201461277902126312255859375;0.1964824017927586374820947412445093505084514617919921875]
      mask Display: e = 0.06;c1 = [120 150 230]/255;c2 = ([120 150 230]+0)/383;c3 = ([120 150 230]+128)/383;patch([0 1 1 0],[0 0 1 1],c1);patch([0 1 1 1-e 1-e 0+e],[0 0 1 1-e 0+e 0+e],c2);patch([0 0 1 1-e 0+e 0+e],[0 1 1 1-e 1-e 0+e],c3);plot([0 1 1 0 0],[0 0 1 1 0]);disp('Weights');
  "IW{1,2}(2,:)'" : Constant  Value=[-0.0204945748265934028775614450523789855651557445526123046875;1.9312316925216492791150812990963459014892578125;-0.349380909352063617756556368476594798266887664794921875;-0.495796724108398423336296900743036530911922454833984375;0.446205717562955295196758243037038482725620269775390625;0.262472904500300974195425851576146669685840606689453125;-0.41517043024050115374024017000920139253139495849609375;0.278255143027667350974496685012127272784709930419921875;-0.58721155899074073403198781306855380535125732421875;-0.31111504995260885753083357485593296587467193603515625;0.2082156225331104615339228303128038533031940460205078125;0.06714824204430365484075338144975830800831317901611328125;-0.2577729533224426550219732234836556017398834228515625;-0.22302526384316123664319775343756191432476043701171875;-0.022003728674898470618614965133019722998142242431640625;0.0647970694014321224596386628036270849406719207763671875;0.121653698494545381425524510632385499775409698486328125;0.032225768311224568807293877625852474011480808258056640625;-0.0749351280816741571744188377124373801052570343017578125;-0.0830815730742837377231779782960074953734874725341796875]
      mask Display: e = 0.06;c1 = [120 150 230]/255;c2 = ([120 150 230]+0)/383;c3 = ([120 150 230]+128)/383;patch([0 1 1 0],[0 0 1 1],c1);patch([0 1 1 1-e 1-e 0+e],[0 0 1 1-e 0+e 0+e],c2);patch([0 0 1 1-e 0+e 0+e],[0 1 1 1-e 1-e 0+e],c3);plot([0 1 1 0 0],[0 0 1 1 0]);disp('Weights');
  "IW{1,2}(3,:)'" : Constant  Value=[0.311296639071176162172349677348393015563488006591796875;0.344762228671464610041397236273041926324367523193359375;0.0278297350072136233378738978672117809765040874481201171875;0.225855871469414937191544368033646605908870697021484375;-0.50201215734075166352567975991405546665191650390625;-0.51006517344202284558463134089834056794643402099609375;0.368850413907754026698881943957530893385410308837890625;-0.401790121272149580722299333501723594963550567626953125;0.32114224203135532942354757324210368096828460693359375;-1.1663541493134153004262998365447856485843658447265625;-0.1478022319722895050464472888052114285528659820556640625;-0.183510303176730615870582141724298708140850067138671875;-0.07367633664230362200431301289427210576832294464111328125;0.1623557999960706654807296445142128504812717437744140625;-0.11271509011977244585356316974866786040365695953369140625;0.184846754962676163014378971638507209718227386474609375;0.3133439802259381234961210793699137866497039794921875;-0.252519800420523632400460201097303070127964019775390625;-0.221360865491497971202505823384854011237621307373046875;-0.1841812971957616229534693275127210654318332672119140625]
      mask Display: e = 0.06;c1 = [120 150 230]/255;c2 = ([120 150 230]+0)/383;c3 = ([120 150 230]+128)/383;patch([0 1 1 0],[0 0 1 1],c1);patch([0 1 1 1-e 1-e 0+e],[0 0 1 1-e 0+e 0+e],c2);patch([0 0 1 1-e 0+e 0+e],[0 1 1 1-e 1-e 0+e],c3);plot([0 1 1 0 0],[0 0 1 1 0]);disp('Weights');
  "IW{1,2}(4,:)'" : Constant  Value=[-0.057514447860808053103465198319099727086722850799560546875;0.2488193461722778554445767440483905375003814697265625;0.436179108525951431118983236956410109996795654296875;0.62850371404861415935982904557022266089916229248046875;0.360353789899425347442729616886936128139495849609375;0.319649554425117887745955158607102930545806884765625;-0.056141492256935675297935262051396421156823635101318359375;-0.06420819240433393859657229540971457026898860931396484375;-0.298330399071270735422700681738206185400485992431640625;0.316682290222883133790077181402011774480342864990234375;0.300197811943785863864064822337240912020206451416015625;0.65177870612658328486332948159542866051197052001953125;0.731649188826106300354013001197017729282379150390625;0.27621917784086125191578275916981510818004608154296875;0.214795029193491526786630174683523364365100860595703125;-0.07538691746936752868801789873032248578965663909912109375;0.311109736894615684921205911450670100748538970947265625;0.175314958149205224469113773011486046016216278076171875;0.60752070052883466733106843093992210924625396728515625;-0.06656813973898330349943108785737422294914722442626953125]
      mask Display: e = 0.06;c1 = [120 150 230]/255;c2 = ([120 150 230]+0)/383;c3 = ([120 150 230]+128)/383;patch([0 1 1 0],[0 0 1 1],c1);patch([0 1 1 1-e 1-e 0+e],[0 0 1 1-e 0+e 0+e],c2);patch([0 0 1 1-e 0+e 0+e],[0 1 1 1-e 1-e 0+e],c3);plot([0 1 1 0 0],[0 0 1 1 0]);disp('Weights');
  "IW{1,2}(5,:)'" : Constant  Value=[-1.6438076496059796927085017159697599709033966064453125;-0.086324763306777685389903354007401503622531890869140625;-0.09369173695724915262861287601481308229267597198486328125;0.254420292022872585047110760569921694695949554443359375;-0.0540278394423806818114286443233140744268894195556640625;0.025839570314925057459287671690617571584880352020263671875;0.483808839659541300992628976018750108778476715087890625;0.031501150613976132419669085038549383170902729034423828125;0.2459673877565530519806458187304087914526462554931640625;-0.04218305595413256170456151039616088382899761199951171875;-0.311907821939236551411767095487448386847972869873046875;-0.35523913097318005060998302724328823387622833251953125;-0.38021712626112214028495372986071743071079254150390625;-0.362205965454087952526407434561406262218952178955078125;-0.431926131174329486217544626924791373312473297119140625;-0.34764619875349367372763254024903289973735809326171875;-0.1256631148851009849298776543946587480604648590087890625;-0.052109898949633533249414796273413230665028095245361328125;-0.350138247160166005134129818543442524969577789306640625;-0.263729362088069796410394474150962196290493011474609375]
      mask Display: e = 0.06;c1 = [120 150 230]/255;c2 = ([120 150 230]+0)/383;c3 = ([120 150 230]+128)/383;patch([0 1 1 0],[0 0 1 1],c1);patch([0 1 1 1-e 1-e 0+e],[0 0 1 1-e 0+e 0+e],c2);patch([0 0 1 1-e 0+e 0+e],[0 1 1 1-e 1-e 0+e],c3);plot([0 1 1 0 0],[0 0 1 1 0]);disp('Weights');
  "IW{1,2}(6,:)'" : Constant  Value=[-0.126946547161197520470210520215914584696292877197265625;-0.10739417764484891770759844575877650640904903411865234375;1.8210936696847757065853556923684664070606231689453125;0.0805106956973491438844803269603289663791656494140625;0.67265333014620309892706018217722885310649871826171875;0.049347224056254017365841235687184962444007396697998046875;-0.08771465728828066465982971067205653525888919830322265625;-0.386646596389371210999996719692717306315898895263671875;0.0814614951451028967976952799290302209556102752685546875;0.1847692939323535010753829510576906614005565643310546875;0.0975849706023748930672212509307428263127803802490234375;0.2368638783828181104684773572444100864231586456298828125;0.184533481879900096433999578948714770376682281494140625;0.2328044728961049525395310411113314330577850341796875;0.66432886846381211665146793166059069335460662841796875;0.2017848609389918390633056333172135055065155029296875;-0.0681323312013900894701379229445592500269412994384765625;0.33143308198795773389377927742316387593746185302734375;0.11090926884688463716077677645444055087864398956298828125;-0.10537243237728100009320542085333727300167083740234375]
      mask Display: e = 0.06;c1 = [120 150 230]/255;c2 = ([120 150 230]+0)/383;c3 = ([120 150 230]+128)/383;patch([0 1 1 0],[0 0 1 1],c1);patch([0 1 1 1-e 1-e 0+e],[0 0 1 1-e 0+e 0+e],c2);patch([0 0 1 1-e 0+e 0+e],[0 1 1 1-e 1-e 0+e],c3);plot([0 1 1 0 0],[0 0 1 1 0]);disp('Weights');
  "IW{1,2}(7,:)'" : Constant  Value=[0.407045031801934131809872496887692250311374664306640625;0.50594537530523042700991709352820180356502532958984375;-0.006874370035477550024138881923363442183472216129302978515625;0.460101943369063182132094880216754972934722900390625;-0.1843383523793279687996715665576630271971225738525390625;-0.4273468064774779140435612134751863777637481689453125;0.32657684054661662020890844360110349953174591064453125;-0.482887354381933031621798591004335321485996246337890625;-2.598383743213501073654470019391737878322601318359375;0.303423856551292503436201286604045890271663665771484375;-0.402184242667662505965608943370170891284942626953125;0.19897535163832824611773730794084258377552032470703125;0.2179711142478014396228758187135099433362483978271484375;-0.16174796697660875910429467694484628736972808837890625;-0.2007879191744248170703457390118273906409740447998046875;-0.785440000903992352476734595256857573986053466796875;0.283299520184668585098819448830909095704555511474609375;-0.22058409323238736821082284222939051687717437744140625;-0.10221069813239268275761872928342199884355068206787109375;-0.21755351921661569836174976444453932344913482666015625]
      mask Display: e = 0.06;c1 = [120 150 230]/255;c2 = ([120 150 230]+0)/383;c3 = ([120 150 230]+128)/383;patch([0 1 1 0],[0 0 1 1],c1);patch([0 1 1 1-e 1-e 0+e],[0 0 1 1-e 0+e 0+e],c2);patch([0 0 1 1-e 0+e 0+e],[0 1 1 1-e 1-e 0+e],c3);plot([0 1 1 0 0],[0 0 1 1 0]);disp('Weights');
  "IW{1,2}(8,:)'" : Constant  Value=[-0.13894941599945964672002673978568054735660552978515625;-0.19210359160348111640104207253898493945598602294921875;0.023064825387133815193241304086768650449812412261962890625;1.201400733368269246881254730396904051303863525390625;0.32834265774768944812223026019637472927570343017578125;0.52654210812649127060325326965539716184139251708984375;-0.3293914298690354680587688562809489667415618896484375;0.4171875659496253607727567214169539511203765869140625;-0.312627971483171174238435696679516695439815521240234375;0.033794282522205724983432872932098689489066600799560546875;0.0677374026563230813291482945714960806071758270263671875;0.032053071412869955925106779659472522325813770294189453125;0.199296522562057543126456948812119662761688232421875;0.050050256175566194827286636837015976198017597198486328125;0.317245630480036899800921901260153390467166900634765625;0.207265742551407894378456830963841639459133148193359375;-0.045075160924855757482720974849144113250076770782470703125;0.3704121818229546558853826354607008397579193115234375;0.051850875414569286281363247326225973665714263916015625;0.184974201118300041191133686879766173660755157470703125]
      mask Display: e = 0.06;c1 = [120 150 230]/255;c2 = ([120 150 230]+0)/383;c3 = ([120 150 230]+128)/383;patch([0 1 1 0],[0 0 1 1],c1);patch([0 1 1 1-e 1-e 0+e],[0 0 1 1-e 0+e 0+e],c2);patch([0 0 1 1-e 0+e 0+e],[0 1 1 1-e 1-e 0+e],c3);plot([0 1 1 0 0],[0 0 1 1 0]);disp('Weights');
  "IW{1,2}(9,:)'" : Constant  Value=[-0.435001277681425657650748917149030603468418121337890625;-0.2161688784686718600713817295400076545774936676025390625;0.2019963442699870548313612061974708922207355499267578125;-0.15392579474173373466072689552675001323223114013671875;-0.12359328339492926807086092821919010020792484283447265625;0.10924243951800226282156103252418688498437404632568359375;-0.12146217718389272499646125424987985752522945404052734375;0.96693327144510654580500386146013624966144561767578125;-0.480853451383004115715635862216004170477390289306640625;0.525166763786194312757515945122577250003814697265625;0.022650694986053689083949080895763472653925418853759765625;0.042120637528565200990993133700612816028296947479248046875;0.29306435756609394704952364918426610529422760009765625;0.00695295809421735133692976660313433967530727386474609375;-0.412155750806342202618992587304092012345790863037109375;-0.1324752065808597889517983503537834621965885162353515625;0.0226674872105853721093726704793880344368517398834228515625;0.55121351512932381666587389190681278705596923828125;-0.317474846615484640466320342966355383396148681640625;0.10419837802455202135920586670181364752352237701416015625]
      mask Display: e = 0.06;c1 = [120 150 230]/255;c2 = ([120 150 230]+0)/383;c3 = ([120 150 230]+128)/383;patch([0 1 1 0],[0 0 1 1],c1);patch([0 1 1 1-e 1-e 0+e],[0 0 1 1-e 0+e 0+e],c2);patch([0 0 1 1-e 0+e 0+e],[0 1 1 1-e 1-e 0+e],c3);plot([0 1 1 0 0],[0 0 1 1 0]);disp('Weights');
  Mux : Mux  Inputs=10
      mask Display: e = 0.06;c1 = [120 150 230]/255;c2 = ([120 150 230]+0)/383;c3 = ([120 150 230]+128)/383;patch([0 1 1 0],[0 0 1 1],c1);patch([0 1 1 1-e 1-e 0+e],[0 0 1 1-e 0+e 0+e],c2);patch([0 0 1 1-e 0+e 0+e],[0 1 1 1-e 1-e 0+e],c3);plot([0 1 1 0 0],[0 0 1 1 0]);disp('Mux');
  dotprod{1..10} (10 alike) : neural/Weight Functions/dotprod
  "iz{1,2}" : Outport
      mask Display: e = 0.06;c1 = [120 230 180]/255;c2 = ([120 230 180]+0)/(256+128);c3 = ([120 230 180]+128)/(256+128);patch([0 1 1 0],[0 0 1 1],c1);patch([0 1 1 1-e 1-e 0+e],[0 0 1 1-e 0+e 0+e],c2);patch([0 0 1 1-e 0+e 0+e],[0 1 1 1-e 1-e 0+e],c3);plot([0 1 1 0 0],[0 0 1 1 0]);
  wires:
  "IW{1,2}(1,:)'"/1 -> dotprod1/1
  "pd{1,2}"/1 -> dotprod1/2, dotprod2/2, dotprod3/2, dotprod4/2, dotprod5/2, dotprod6/2, dotprod7/2, dotprod8/2, dotprod9/2, dotprod10/2
  dotprod1/1 -> Mux/1
  "IW{1,2}(2,:)'"/1 -> dotprod2/1
  dotprod2/1 -> Mux/2
  "IW{1,2}(3,:)'"/1 -> dotprod3/1
  dotprod3/1 -> Mux/3
  "IW{1,2}(4,:)'"/1 -> dotprod4/1
  dotprod4/1 -> Mux/4
  "IW{1,2}(5,:)'"/1 -> dotprod5/1
  dotprod5/1 -> Mux/5
  "IW{1,2}(6,:)'"/1 -> dotprod6/1
  dotprod6/1 -> Mux/6
  "IW{1,2}(7,:)'"/1 -> dotprod7/1
  dotprod7/1 -> Mux/7
  "IW{1,2}(8,:)'"/1 -> dotprod8/1
  dotprod8/1 -> Mux/8
  "IW{1,2}(9,:)'"/1 -> dotprod9/1
  dotprod9/1 -> Mux/9
  "IW{1,2}(10,:)'"/1 -> dotprod10/1
  dotprod10/1 -> Mux/10
  Mux/1 -> "iz{1,2}"/1

== system untitled/NARX Neural Network/Layer 2/Delays 1 ==
  "p{2}" : Inport  PortDimensions=10  SampleTime=1
      mask Display: e = 0.06;c1 = [120 230 180]/255;c2 = ([120 230 180]+0)/(256+128);c3 = ([120 230 180]+128)/(256+128);patch([0 1 1 0],[0 0 1 1],c1);patch([0 1 1 1-e 1-e 0+e],[0 0 1 1-e 0+e 0+e],c2);patch([0 0 1 1-e 0+e 0+e],[0 1 1 1-e 1-e 0+e],c3);plot([0 1 1 0 0],[0 0 1 1 0]);
  mux : Mux  Inputs=1
      mask Display: e = 0.06;c1 = [120 150 230]/255;c2 = ([120 150 230]+0)/383;c3 = ([120 150 230]+128)/383;patch([0 1 1 0],[0 0 1 1],c1);patch([0 1 1 1-e 1-e 0+e],[0 0 1 1-e 0+e 0+e],c2);patch([0 0 1 1-e 0+e 0+e],[0 1 1 1-e 1-e 0+e],c3);plot([0 1 1 0 0],[0 0 1 1 0]);disp('Mux')
  "pd{2,1}" : Outport
      mask Display: e = 0.06;c1 = [120 230 180]/255;c2 = ([120 230 180]+0)/(256+128);c3 = ([120 230 180]+128)/(256+128);patch([0 1 1 0],[0 0 1 1],c1);patch([0 1 1 1-e 1-e 0+e],[0 0 1 1-e 0+e 0+e],c2);patch([0 0 1 1-e 0+e 0+e],[0 1 1 1-e 1-e 0+e],c3);plot([0 1 1 0 0],[0 0 1 1 0]);
  wires:
  "p{2}"/1 -> mux/1
  mux/1 -> "pd{2,1}"/1
